simulink model "s_c107m32k_vlbi"  (R2018a)
(part 22 of 201)

      |     mask_enables{ismember(mask_names, 'sample_period')} = 'on';
      | end
      | set_param(gcb, 'MaskEnables', mask_enables);
      mask DialogControl ParameterTabVar0 Prompt: Setup
  sync_latch_hmc_wradd : Subsystem  Tag=xps:sw_reg  Commented=on  AncestorBlock=xps_library/Memory/software_register  mask(swreg){io_dir=To Processor, io_delay=0, init_val=0, sample_period=1, names=count, bitwidths=27, bin_pts=0, arith_types=0, sim_port=off, show_format=on}
      mask prompts: io_dir "I/O direction"; io_delay "I/O delay"; init_val "Initial Value"; sample_period "Sample period"; names "Bitfield names [msb...lsb]"; bitwidths "Bitfield widths"; bin_pts "Bitfield binary pts"; arith_types "Bitfield types, ufix=0, fix=1, bool=2"; sim_port "Provide sim input/output?"; show_format "Print format string?"
      mask help: A 32-bit software-accessible register. Can be divided into bitfields of varying widths and types using the fields in the block mask.
      mask init:
      | swreg_init(gcb)
      settings: AttributesFormatString=1output:uf27.0 = 27 bits
      mask TypeOptions io_dir: To Processor | From Processor
      mask Callback io_dir:
      | mask_enables = get_param(gcb, 'MaskEnables');
      | mask_names = get_param(gcb, 'MaskNames');
      | if strcmp(get_param(gcb, 'io_dir'), 'To Processor'),
      |     mask_enables{ismember(mask_names, 'sample_period')} = 'off';
      | else
      |     mask_enables{ismember(mask_names, 'sample_period')} = 'on';
      | end
      | set_param(gcb, 'MaskEnables', mask_enables);
      mask DialogControl ParameterTabVar0 Prompt: Setup
  sync_time_hmc_in_lsw : Subsystem  Tag=xps:sw_reg  Commented=on  AncestorBlock=xps_library/Memory/software_register  mask(swreg){io_dir=To Processor, io_delay=0, init_val=0, sample_period=1, names=lsw, bitwidths=32, bin_pts=0, arith_types=0, sim_port=off, show_format=on}
      mask prompts: io_dir "I/O direction"; io_delay "I/O delay"; init_val "Initial Value"; sample_period "Sample period"; names "Bitfield names [msb...lsb]"; bitwidths "Bitfield widths"; bin_pts "Bitfield binary pts"; arith_types "Bitfield types, ufix=0, fix=1, bool=2"; sim_port "Provide sim input/output?"; show_format "Print format string?"
      mask help: A 32-bit software-accessible register. Can be divided into bitfields of varying widths and types using the fields in the block mask.
      mask init:
      | swreg_init(gcb)
      settings: AttributesFormatString=1output:uf32.0 = 32 bits
      mask TypeOptions io_dir: To Processor | From Processor
      mask Callback io_dir:
      | mask_enables = get_param(gcb, 'MaskEnables');
      | mask_names = get_param(gcb, 'MaskNames');
      | if strcmp(get_param(gcb, 'io_dir'), 'To Processor'),
      |     mask_enables{ismember(mask_names, 'sample_period')} = 'off';
      | else
      |     mask_enables{ismember(mask_names, 'sample_period')} = 'on';
      | end
      | set_param(gcb, 'MaskEnables', mask_enables);
      mask DialogControl ParameterTabVar0 Prompt: Setup
  sync_time_hmc_in_msw : Subsystem  Tag=xps:sw_reg  Commented=on  AncestorBlock=xps_library/Memory/software_register  mask(swreg){io_dir=To Processor, io_delay=0, init_val=0, sample_period=1, names=msw, bitwidths=16, bin_pts=0, arith_types=0, sim_port=off, show_format=on}
      mask prompts: io_dir "I/O direction"; io_delay "I/O delay"; init_val "Initial Value"; sample_period "Sample period"; names "Bitfield names [msb...lsb]"; bitwidths "Bitfield widths"; bin_pts "Bitfield binary pts"; arith_types "Bitfield types, ufix=0, fix=1, bool=2"; sim_port "Provide sim input/output?"; show_format "Print format string?"
      mask help: A 32-bit software-accessible register. Can be divided into bitfields of varying widths and types using the fields in the block mask.
      mask init:
      | swreg_init(gcb)
      settings: AttributesFormatString=1output:uf16.0 = 16 bits
      mask TypeOptions io_dir: To Processor | From Processor
      mask Callback io_dir:
      | mask_enables = get_param(gcb, 'MaskEnables');
      | mask_names = get_param(gcb, 'MaskNames');
      | if strcmp(get_param(gcb, 'io_dir'), 'To Processor'),
      |     mask_enables{ismember(mask_names, 'sample_period')} = 'off';
      | else
      |     mask_enables{ismember(mask_names, 'sample_period')} = 'on';
      | end
      | set_param(gcb, 'MaskEnables', mask_enables);
      mask DialogControl ParameterTabVar0 Prompt: Setup
  sync_time_hmc_out_lsw : Subsystem  Tag=xps:sw_reg  Commented=on  AncestorBlock=xps_library/Memory/software_register  mask(swreg){io_dir=To Processor, io_delay=0, init_val=0, sample_period=1, names=lsw, bitwidths=32, bin_pts=0, arith_types=0, sim_port=off, show_format=on}
      mask prompts: io_dir "I/O direction"; io_delay "I/O delay"; init_val "Initial Value"; sample_period "Sample period"; names "Bitfield names [msb...lsb]"; bitwidths "Bitfield widths"; bin_pts "Bitfield binary pts"; arith_types "Bitfield types, ufix=0, fix=1, bool=2"; sim_port "Provide sim input/output?"; show_format "Print format string?"
      mask help: A 32-bit software-accessible register. Can be divided into bitfields of varying widths and types using the fields in the block mask.
      mask init:
      | swreg_init(gcb)
      settings: AttributesFormatString=1output:uf32.0 = 32 bits
      mask TypeOptions io_dir: To Processor | From Processor
      mask Callback io_dir:
      | mask_enables = get_param(gcb, 'MaskEnables');
      | mask_names = get_param(gcb, 'MaskNames');
      | if strcmp(get_param(gcb, 'io_dir'), 'To Processor'),
      |     mask_enables{ismember(mask_names, 'sample_period')} = 'off';
      | else
      |     mask_enables{ismember(mask_names, 'sample_period')} = 'on';
      | end
      | set_param(gcb, 'MaskEnables', mask_enables);
      mask DialogControl ParameterTabVar0 Prompt: Setup
  sync_time_hmc_out_msw : Subsystem  Tag=xps:sw_reg  Commented=on  AncestorBlock=xps_library/Memory/software_register  mask(swreg){io_dir=To Processor, io_delay=0, init_val=0, sample_period=1, names=msw, bitwidths=16, bin_pts=0, arith_types=0, sim_port=off, show_format=on}
      mask prompts: io_dir "I/O direction"; io_delay "I/O delay"; init_val "Initial Value"; sample_period "Sample period"; names "Bitfield names [msb...lsb]"; bitwidths "Bitfield widths"; bin_pts "Bitfield binary pts"; arith_types "Bitfield types, ufix=0, fix=1, bool=2"; sim_port "Provide sim input/output?"; show_format "Print format string?"
      mask help: A 32-bit software-accessible register. Can be divided into bitfields of varying widths and types using the fields in the block mask.
      mask init:
      | swreg_init(gcb)
      settings: AttributesFormatString=1output:uf16.0 = 16 bits
      mask TypeOptions io_dir: To Processor | From Processor
      mask Callback io_dir:
      | mask_enables = get_param(gcb, 'MaskEnables');
      | mask_names = get_param(gcb, 'MaskNames');
      | if strcmp(get_param(gcb, 'io_dir'), 'To Processor'),
      |     mask_enables{ismember(mask_names, 'sample_period')} = 'off';
      | else
      |     mask_enables{ismember(mask_names, 'sample_period')} = 'on';
      | end
      | set_param(gcb, 'MaskEnables', mask_enables);
      mask DialogControl ParameterTabVar0 Prompt: Setup
  time_gen_1 : Subsystem  Commented=on  mask{n_bits_period=0, n_bits_increment=3, n_bits_counter=48}
      mask prompts: n_bits_period "Period (2^?)"; n_bits_increment "Increment (2^?)"; n_bits_counter "Counter size (2^?)"
  time_gen_3 : Subsystem  Commented=on  mask{n_bits_period=0, n_bits_increment=3, n_bits_counter=48}
      mask prompts: n_bits_period "Period (2^?)"; n_bits_increment "Increment (2^?)"; n_bits_counter "Counter size (2^?)"
  tvg_data_gen1 : Subsystem
  tvg_data_gen_oneshot : Subsystem
      mask Display:
      | color('red');
      | disp('ONE SHOT!!');
      | % color('green');
      | % port_label('input', 1, 'dv')
      | % color('red');
      | % port_label('output', 1, 'err')
  tvg_data_tone_gen : Subsystem
  tvg_data_tone_gen1 : Subsystem
  tvg_freq_ramp_gen0 : Subsystem
  tvg_freq_ramp_gen1 : Subsystem
  tvg_time_ramp_gen0 : Subsystem
  we_delay1 : Subsystem  Tag=cmac_delinked  Commented=on  mask(pipeline){csp_latency=2}
      mask prompts: csp_latency "Latency"
      mask help:
      | An explicitly laid-out delay line to avoid mapping to SRL16s
      | for use in pipelining to help achieve timing closure.
      mask init:
      | pipeline_init(gcb,'latency',csp_latency);
      settings: AttributesFormatString=Latency = %<latency>
      mask Display:
      | port_label('input', 1, 'd');
      | port_label('output', 1, 'q');
      | disp(['Z^-', num2str(csp_latency)]);
  we_delay10 : Subsystem  Tag=cmac_delinked  Commented=on  mask(pipeline){csp_latency=2}
      mask prompts: csp_latency "Latency"
      mask help:
      | An explicitly laid-out delay line to avoid mapping to SRL16s
      | for use in pipelining to help achieve timing closure.
      mask init:
      | pipeline_init(gcb,'latency',csp_latency);
      settings: AttributesFormatString=Latency = %<latency>
      mask Display:
      | port_label('input', 1, 'd');
      | port_label('output', 1, 'q');
      | disp(['Z^-', num2str(csp_latency)]);
  we_delay11 : Subsystem  Tag=cmac_delinked  Commented=on  mask(pipeline){csp_latency=2}
      mask prompts: csp_latency "Latency"
      mask help:
      | An explicitly laid-out delay line to avoid mapping to SRL16s
      | for use in pipelining to help achieve timing closure.
      mask init:
      | pipeline_init(gcb,'latency',csp_latency);
      settings: AttributesFormatString=Latency = %<latency>
      mask Display:
      | port_label('input', 1, 'd');
      | port_label('output', 1, 'q');
      | disp(['Z^-', num2str(csp_latency)]);
  we_delay12 : Subsystem  Tag=cmac_delinked  Commented=on  mask(pipeline){csp_latency=2}
      mask prompts: csp_latency "Latency"
      mask help:
      | An explicitly laid-out delay line to avoid mapping to SRL16s
      | for use in pipelining to help achieve timing closure.
      mask init:
      | pipeline_init(gcb,'latency',csp_latency);
      settings: AttributesFormatString=Latency = %<latency>
      mask Display:
      | port_label('input', 1, 'd');
      | port_label('output', 1, 'q');
      | disp(['Z^-', num2str(csp_latency)]);
  we_delay13 : Subsystem  Tag=cmac_delinked  Commented=on  mask(pipeline){csp_latency=2}
      mask prompts: csp_latency "Latency"
      mask help:
      | An explicitly laid-out delay line to avoid mapping to SRL16s
      | for use in pipelining to help achieve timing closure.
      mask init:
      | pipeline_init(gcb,'latency',csp_latency);
      settings: AttributesFormatString=Latency = %<latency>
      mask Display:
      | port_label('input', 1, 'd');
      | port_label('output', 1, 'q');
      | disp(['Z^-', num2str(csp_latency)]);
  we_delay14 : Subsystem  Tag=cmac_delinked  Commented=on  mask(pipeline){csp_latency=2}
      mask prompts: csp_latency "Latency"
      mask help:
      | An explicitly laid-out delay line to avoid mapping to SRL16s
      | for use in pipelining to help achieve timing closure.
      mask init:
      | pipeline_init(gcb,'latency',csp_latency);
      settings: AttributesFormatString=Latency = %<latency>
      mask Display:
      | port_label('input', 1, 'd');
      | port_label('output', 1, 'q');
      | disp(['Z^-', num2str(csp_latency)]);
  we_delay15 : Subsystem  Tag=cmac_delinked  Commented=on  mask(pipeline){csp_latency=2}
      mask prompts: csp_latency "Latency"
      mask help:
      | An explicitly laid-out delay line to avoid mapping to SRL16s
      | for use in pipelining to help achieve timing closure.
      mask init:
      | pipeline_init(gcb,'latency',csp_latency);
      settings: AttributesFormatString=Latency = %<latency>
      mask Display:
      | port_label('input', 1, 'd');
      | port_label('output', 1, 'q');
      | disp(['Z^-', num2str(csp_latency)]);
  we_delay16 : Subsystem  Tag=cmac_delinked  Commented=on  mask(pipeline){csp_latency=2}
      mask prompts: csp_latency "Latency"
      mask help:
      | An explicitly laid-out delay line to avoid mapping to SRL16s
      | for use in pipelining to help achieve timing closure.
      mask init:
      | pipeline_init(gcb,'latency',csp_latency);
      settings: AttributesFormatString=Latency = %<latency>
      mask Display:
      | port_label('input', 1, 'd');
      | port_label('output', 1, 'q');
      | disp(['Z^-', num2str(csp_latency)]);
  we_delay17 : Subsystem  Tag=cmac_delinked  Commented=on  mask(pipeline){csp_latency=2}
      mask prompts: csp_latency "Latency"
      mask help:
      | An explicitly laid-out delay line to avoid mapping to SRL16s
      | for use in pipelining to help achieve timing closure.
      mask init:
      | pipeline_init(gcb,'latency',csp_latency);
      settings: AttributesFormatString=Latency = %<latency>
      mask Display:
      | port_label('input', 1, 'd');
      | port_label('output', 1, 'q');
      | disp(['Z^-', num2str(csp_latency)]);
  we_delay18 : Subsystem  Tag=cmac_delinked  Commented=on  mask(pipeline){csp_latency=2}
      mask prompts: csp_latency "Latency"
      mask help:
      | An explicitly laid-out delay line to avoid mapping to SRL16s
      | for use in pipelining to help achieve timing closure.
      mask init:
      | pipeline_init(gcb,'latency',csp_latency);
      settings: AttributesFormatString=Latency = %<latency>
      mask Display:
      | port_label('input', 1, 'd');
      | port_label('output', 1, 'q');
      | disp(['Z^-', num2str(csp_latency)]);
  we_delay19 : Subsystem  Tag=cmac_delinked  Commented=on  mask(pipeline){csp_latency=2}
      mask prompts: csp_latency "Latency"
      mask help:
      | An explicitly laid-out delay line to avoid mapping to SRL16s
      | for use in pipelining to help achieve timing closure.
      mask init:
      | pipeline_init(gcb,'latency',csp_latency);
      settings: AttributesFormatString=Latency = %<latency>
      mask Display:
      | port_label('input', 1, 'd');
      | port_label('output', 1, 'q');
      | disp(['Z^-', num2str(csp_latency)]);
  we_delay2 : Subsystem  Tag=cmac_delinked  Commented=on  mask(pipeline){csp_latency=2}
      mask prompts: csp_latency "Latency"
      mask help:
      | An explicitly laid-out delay line to avoid mapping to SRL16s
      | for use in pipelining to help achieve timing closure.
      mask init:
      | pipeline_init(gcb,'latency',csp_latency);
      settings: AttributesFormatString=Latency = %<latency>
      mask Display:
      | port_label('input', 1, 'd');
      | port_label('output', 1, 'q');
      | disp(['Z^-', num2str(csp_latency)]);
  we_delay20 : Subsystem  Tag=cmac_delinked  Commented=on  mask(pipeline){csp_latency=2}
      mask prompts: csp_latency "Latency"
      mask help:
      | An explicitly laid-out delay line to avoid mapping to SRL16s
      | for use in pipelining to help achieve timing closure.
      mask init:
      | pipeline_init(gcb,'latency',csp_latency);
      settings: AttributesFormatString=Latency = %<latency>
      mask Display:
      | port_label('input', 1, 'd');
      | port_label('output', 1, 'q');
      | disp(['Z^-', num2str(csp_latency)]);
  we_delay21 : Subsystem  Tag=cmac_delinked  Commented=on  mask(pipeline){csp_latency=2}
      mask prompts: csp_latency "Latency"
      mask help:
      | An explicitly laid-out delay line to avoid mapping to SRL16s
      | for use in pipelining to help achieve timing closure.
      mask init:
      | pipeline_init(gcb,'latency',csp_latency);
      settings: AttributesFormatString=Latency = %<latency>
      mask Display:
      | port_label('input', 1, 'd');
      | port_label('output', 1, 'q');
      | disp(['Z^-', num2str(csp_latency)]);
  we_delay22 : Subsystem  Tag=cmac_delinked  Commented=on  mask(pipeline){csp_latency=2}
      mask prompts: csp_latency "Latency"
      mask help:
      | An explicitly laid-out delay line to avoid mapping to SRL16s
      | for use in pipelining to help achieve timing closure.
      mask init:
      | pipeline_init(gcb,'latency',csp_latency);
      settings: AttributesFormatString=Latency = %<latency>
      mask Display:
      | port_label('input', 1, 'd');
      | port_label('output', 1, 'q');
      | disp(['Z^-', num2str(csp_latency)]);
  we_delay23 : Subsystem  Tag=cmac_delinked  Commented=on  mask(pipeline){csp_latency=2}
      mask prompts: csp_latency "Latency"
      mask help:
      | An explicitly laid-out delay line to avoid mapping to SRL16s
      | for use in pipelining to help achieve timing closure.
      mask init:
      | pipeline_init(gcb,'latency',csp_latency);
      settings: AttributesFormatString=Latency = %<latency>
      mask Display:
      | port_label('input', 1, 'd');
      | port_label('output', 1, 'q');
      | disp(['Z^-', num2str(csp_latency)]);
  we_delay24 : Subsystem  Tag=cmac_delinked  Commented=on  mask(pipeline){csp_latency=2}
      mask prompts: csp_latency "Latency"
      mask help:
      | An explicitly laid-out delay line to avoid mapping to SRL16s
      | for use in pipelining to help achieve timing closure.
      mask init:
      | pipeline_init(gcb,'latency',csp_latency);
      settings: AttributesFormatString=Latency = %<latency>
      mask Display:
      | port_label('input', 1, 'd');
      | port_label('output', 1, 'q');
      | disp(['Z^-', num2str(csp_latency)]);
  we_delay25 : Subsystem  Tag=cmac_delinked  Commented=on  mask(pipeline){csp_latency=2}
      mask prompts: csp_latency "Latency"
      mask help:
      | An explicitly laid-out delay line to avoid mapping to SRL16s
      | for use in pipelining to help achieve timing closure.
      mask init:
      | pipeline_init(gcb,'latency',csp_latency);
      settings: AttributesFormatString=Latency = %<latency>
      mask Display:
      | port_label('input', 1, 'd');
      | port_label('output', 1, 'q');
      | disp(['Z^-', num2str(csp_latency)]);
  we_delay26 : Subsystem  Tag=cmac_delinked  Commented=on  mask(pipeline){csp_latency=2}
      mask prompts: csp_latency "Latency"
      mask help:
      | An explicitly laid-out delay line to avoid mapping to SRL16s
      | for use in pipelining to help achieve timing closure.
      mask init:
      | pipeline_init(gcb,'latency',csp_latency);
      settings: AttributesFormatString=Latency = %<latency>
      mask Display:
      | port_label('input', 1, 'd');
      | port_label('output', 1, 'q');
      | disp(['Z^-', num2str(csp_latency)]);
  we_delay27 : Subsystem  Tag=cmac_delinked  Commented=on  mask(pipeline){csp_latency=2}
      mask prompts: csp_latency "Latency"
      mask help:
      | An explicitly laid-out delay line to avoid mapping to SRL16s
      | for use in pipelining to help achieve timing closure.
      mask init:
      | pipeline_init(gcb,'latency',csp_latency);
      settings: AttributesFormatString=Latency = %<latency>
      mask Display:
      | port_label('input', 1, 'd');
      | port_label('output', 1, 'q');
      | disp(['Z^-', num2str(csp_latency)]);
  we_delay28 : Subsystem  Tag=cmac_delinked  Commented=on  mask(pipeline){csp_latency=2}
      mask prompts: csp_latency "Latency"
      mask help:
      | An explicitly laid-out delay line to avoid mapping to SRL16s
      | for use in pipelining to help achieve timing closure.
      mask init:
      | pipeline_init(gcb,'latency',csp_latency);
      settings: AttributesFormatString=Latency = %<latency>
      mask Display:
      | port_label('input', 1, 'd');
      | port_label('output', 1, 'q');
      | disp(['Z^-', num2str(csp_latency)]);
  we_delay29 : Subsystem  Tag=cmac_delinked  Commented=on  mask(pipeline){csp_latency=2}
      mask prompts: csp_latency "Latency"
      mask help:
      | An explicitly laid-out delay line to avoid mapping to SRL16s
      | for use in pipelining to help achieve timing closure.
      mask init:
      | pipeline_init(gcb,'latency',csp_latency);
      settings: AttributesFormatString=Latency = %<latency>
      mask Display:
      | port_label('input', 1, 'd');
      | port_label('output', 1, 'q');
      | disp(['Z^-', num2str(csp_latency)]);
  we_delay3 : Subsystem  Tag=cmac_delinked  Commented=on  mask(pipeline){csp_latency=2}
      mask prompts: csp_latency "Latency"
      mask help:
      | An explicitly laid-out delay line to avoid mapping to SRL16s
      | for use in pipelining to help achieve timing closure.
      mask init:
      | pipeline_init(gcb,'latency',csp_latency);
      settings: AttributesFormatString=Latency = %<latency>
      mask Display:
      | port_label('input', 1, 'd');
      | port_label('output', 1, 'q');
      | disp(['Z^-', num2str(csp_latency)]);
  we_delay30 : Subsystem  Tag=cmac_delinked  Commented=on  mask(pipeline){csp_latency=2}
      mask prompts: csp_latency "Latency"
      mask help:
      | An explicitly laid-out delay line to avoid mapping to SRL16s
      | for use in pipelining to help achieve timing closure.
      mask init:
      | pipeline_init(gcb,'latency',csp_latency);
      settings: AttributesFormatString=Latency = %<latency>
      mask Display:
      | port_label('input', 1, 'd');
      | port_label('output', 1, 'q');
      | disp(['Z^-', num2str(csp_latency)]);
  we_delay31 : Subsystem  Tag=cmac_delinked  Commented=on  mask(pipeline){csp_latency=2}
      mask prompts: csp_latency "Latency"
      mask help:
      | An explicitly laid-out delay line to avoid mapping to SRL16s
      | for use in pipelining to help achieve timing closure.
      mask init:
      | pipeline_init(gcb,'latency',csp_latency);
      settings: AttributesFormatString=Latency = %<latency>
      mask Display:
      | port_label('input', 1, 'd');
      | port_label('output', 1, 'q');
      | disp(['Z^-', num2str(csp_latency)]);
  we_delay32 : Subsystem  Tag=cmac_delinked  Commented=on  mask(pipeline){csp_latency=2}
      mask prompts: csp_latency "Latency"
      mask help:
      | An explicitly laid-out delay line to avoid mapping to SRL16s
      | for use in pipelining to help achieve timing closure.
      mask init:
      | pipeline_init(gcb,'latency',csp_latency);
      settings: AttributesFormatString=Latency = %<latency>
      mask Display:
      | port_label('input', 1, 'd');
      | port_label('output', 1, 'q');
      | disp(['Z^-', num2str(csp_latency)]);
  we_delay33 : Subsystem  Tag=cmac_delinked  Commented=on  mask(pipeline){csp_latency=2}
      mask prompts: csp_latency "Latency"
      mask help:
      | An explicitly laid-out delay line to avoid mapping to SRL16s
      | for use in pipelining to help achieve timing closure.
      mask init:
      | pipeline_init(gcb,'latency',csp_latency);
      settings: AttributesFormatString=Latency = %<latency>
      mask Display:
      | port_label('input', 1, 'd');
      | port_label('output', 1, 'q');
      | disp(['Z^-', num2str(csp_latency)]);
  we_delay34 : Subsystem  Tag=cmac_delinked  Commented=on  mask(pipeline){csp_latency=2}
      mask prompts: csp_latency "Latency"
      mask help:
      | An explicitly laid-out delay line to avoid mapping to SRL16s
      | for use in pipelining to help achieve timing closure.
      mask init:
      | pipeline_init(gcb,'latency',csp_latency);
      settings: AttributesFormatString=Latency = %<latency>
      mask Display:
      | port_label('input', 1, 'd');
      | port_label('output', 1, 'q');
      | disp(['Z^-', num2str(csp_latency)]);
  we_delay35 : Subsystem  Tag=cmac_delinked  Commented=on  mask(pipeline){csp_latency=2}
      mask prompts: csp_latency "Latency"
      mask help:
      | An explicitly laid-out delay line to avoid mapping to SRL16s
      | for use in pipelining to help achieve timing closure.
      mask init:
      | pipeline_init(gcb,'latency',csp_latency);
      settings: AttributesFormatString=Latency = %<latency>
      mask Display:
      | port_label('input', 1, 'd');
      | port_label('output', 1, 'q');
      | disp(['Z^-', num2str(csp_latency)]);
  we_delay36 : Subsystem  Tag=cmac_delinked  Commented=on  mask(pipeline){csp_latency=2}
      mask prompts: csp_latency "Latency"
      mask help:
      | An explicitly laid-out delay line to avoid mapping to SRL16s
      | for use in pipelining to help achieve timing closure.
      mask init:
      | pipeline_init(gcb,'latency',csp_latency);
      settings: AttributesFormatString=Latency = %<latency>
      mask Display:
      | port_label('input', 1, 'd');
      | port_label('output', 1, 'q');
      | disp(['Z^-', num2str(csp_latency)]);
  we_delay37 : Subsystem  Tag=cmac_delinked  Commented=on  mask(pipeline){csp_latency=2}
      mask prompts: csp_latency "Latency"
      mask help:
      | An explicitly laid-out delay line to avoid mapping to SRL16s
      | for use in pipelining to help achieve timing closure.
      mask init:
      | pipeline_init(gcb,'latency',csp_latency);
      settings: AttributesFormatString=Latency = %<latency>
      mask Display:
      | port_label('input', 1, 'd');
      | port_label('output', 1, 'q');
      | disp(['Z^-', num2str(csp_latency)]);
  we_delay38 : Subsystem  Tag=cmac_delinked  Commented=on  mask(pipeline){csp_latency=2}
      mask prompts: csp_latency "Latency"
      mask help:
      | An explicitly laid-out delay line to avoid mapping to SRL16s
      | for use in pipelining to help achieve timing closure.
      mask init:
      | pipeline_init(gcb,'latency',csp_latency);
      settings: AttributesFormatString=Latency = %<latency>
      mask Display:
      | port_label('input', 1, 'd');
      | port_label('output', 1, 'q');
      | disp(['Z^-', num2str(csp_latency)]);
  we_delay39 : Subsystem  Tag=cmac_delinked  Commented=on  mask(pipeline){csp_latency=2}
      mask prompts: csp_latency "Latency"
      mask help:
      | An explicitly laid-out delay line to avoid mapping to SRL16s
      | for use in pipelining to help achieve timing closure.
      mask init:
      | pipeline_init(gcb,'latency',csp_latency);
      settings: AttributesFormatString=Latency = %<latency>
      mask Display:
      | port_label('input', 1, 'd');
      | port_label('output', 1, 'q');
      | disp(['Z^-', num2str(csp_latency)]);
  we_delay4 : Subsystem  Tag=cmac_delinked  Commented=on  mask(pipeline){csp_latency=2}
      mask prompts: csp_latency "Latency"
      mask help:
      | An explicitly laid-out delay line to avoid mapping to SRL16s
      | for use in pipelining to help achieve timing closure.
      mask init:
      | pipeline_init(gcb,'latency',csp_latency);
      settings: AttributesFormatString=Latency = %<latency>
      mask Display:
      | port_label('input', 1, 'd');
      | port_label('output', 1, 'q');
      | disp(['Z^-', num2str(csp_latency)]);
  we_delay5 : Subsystem  Tag=cmac_delinked  Commented=on  mask(pipeline){csp_latency=2}
      mask prompts: csp_latency "Latency"
      mask help:
      | An explicitly laid-out delay line to avoid mapping to SRL16s
      | for use in pipelining to help achieve timing closure.
      mask init:
      | pipeline_init(gcb,'latency',csp_latency);
      settings: AttributesFormatString=Latency = %<latency>
      mask Display:
      | port_label('input', 1, 'd');
      | port_label('output', 1, 'q');
      | disp(['Z^-', num2str(csp_latency)]);
  we_delay53 : Subsystem  Tag=cmac_delinked  Commented=on  mask(pipeline){csp_latency=2}
      mask prompts: csp_latency "Latency"
      mask help:
      | An explicitly laid-out delay line to avoid mapping to SRL16s
      | for use in pipelining to help achieve timing closure.
      mask init:
      | pipeline_init(gcb,'latency',csp_latency);
      settings: AttributesFormatString=Latency = %<latency>
      mask Display:
      | port_label('input', 1, 'd');
      | port_label('output', 1, 'q');
      | disp(['Z^-', num2str(csp_latency)]);
  we_delay6 : Subsystem  Tag=cmac_delinked  Commented=on  mask(pipeline){csp_latency=2}
      mask prompts: csp_latency "Latency"
      mask help:
      | An explicitly laid-out delay line to avoid mapping to SRL16s
      | for use in pipelining to help achieve timing closure.
      mask init:
      | pipeline_init(gcb,'latency',csp_latency);
      settings: AttributesFormatString=Latency = %<latency>
      mask Display:
      | port_label('input', 1, 'd');
      | port_label('output', 1, 'q');
      | disp(['Z^-', num2str(csp_latency)]);
  we_delay66 : Subsystem  Tag=cmac_delinked  Commented=on  mask(pipeline){csp_latency=2}
      mask prompts: csp_latency "Latency"
      mask help:
      | An explicitly laid-out delay line to avoid mapping to SRL16s
      | for use in pipelining to help achieve timing closure.
      mask init:
      | pipeline_init(gcb,'latency',csp_latency);
      settings: AttributesFormatString=Latency = %<latency>
      mask Display:
      | port_label('input', 1, 'd');
      | port_label('output', 1, 'q');
      | disp(['Z^-', num2str(csp_latency)]);
  we_delay7 : Subsystem  Tag=cmac_delinked  Commented=on  mask(pipeline){csp_latency=2}
      mask prompts: csp_latency "Latency"
      mask help:
      | An explicitly laid-out delay line to avoid mapping to SRL16s
      | for use in pipelining to help achieve timing closure.
      mask init:
      | pipeline_init(gcb,'latency',csp_latency);
      settings: AttributesFormatString=Latency = %<latency>
      mask Display:
      | port_label('input', 1, 'd');
      | port_label('output', 1, 'q');
      | disp(['Z^-', num2str(csp_latency)]);
  we_delay8 : Subsystem  Tag=cmac_delinked  Commented=on  mask(pipeline){csp_latency=2}
      mask prompts: csp_latency "Latency"
      mask help:
      | An explicitly laid-out delay line to avoid mapping to SRL16s
      | for use in pipelining to help achieve timing closure.
      mask init:
      | pipeline_init(gcb,'latency',csp_latency);
      settings: AttributesFormatString=Latency = %<latency>
      mask Display:
      | port_label('input', 1, 'd');
      | port_label('output', 1, 'q');
      | disp(['Z^-', num2str(csp_latency)]);
  we_delay9 : Subsystem  Tag=cmac_delinked  Commented=on  mask(pipeline){csp_latency=2}
      mask prompts: csp_latency "Latency"
      mask help:
      | An explicitly laid-out delay line to avoid mapping to SRL16s
      | for use in pipelining to help achieve timing closure.
      mask init:
      | pipeline_init(gcb,'latency',csp_latency);
      settings: AttributesFormatString=Latency = %<latency>
      mask Display:
      | port_label('input', 1, 'd');
      | port_label('output', 1, 'q');
      | disp(['Z^-', num2str(csp_latency)]);
  xeng_match : Subsystem  Tag=xps:sw_reg  AncestorBlock=xps_library/Memory/software_register  mask(swreg){io_dir=From Processor, io_delay=0, init_val=0, sample_period=1, names=[val], bitwidths=[3], bin_pts=0, arith_types=0, sim_port=on, show_format=on}
      mask prompts: io_dir "I/O direction"; io_delay "I/O delay"; init_val "Initial Value"; sample_period "Sample period"; names "Bitfield names [msb...lsb]"; bitwidths "Bitfield widths"; bin_pts "Bitfield binary pts"; arith_types "Bitfield types, ufix=0, fix=1, bool=2"; sim_port "Provide sim input/output?"; show_format "Print format string?"
      mask help: A 32-bit software-accessible register. Can be divided into bitfields of varying widths and types using the fields in the block mask.
      mask init:
      | swreg_init(gcb)
      settings: AttributesFormatString=1input:uf3.0 = 3 bits
      mask TypeOptions io_dir: To Processor | From Processor
      mask Callback io_dir:
      | mask_enables = get_param(gcb, 'MaskEnables');
      | mask_names = get_param(gcb, 'MaskNames');
      | if strcmp(get_param(gcb, 'io_dir'), 'To Processor'),
      |     mask_enables{ismember(mask_names, 'sample_period')} = 'off';
      | else
      |     mask_enables{ismember(mask_names, 'sample_period')} = 'on';
      | end
      | set_param(gcb, 'MaskEnables', mask_enables);
      mask DialogControl ParameterTabVar0 Prompt: Setup
  xidx_trig_thresh : Subsystem  Tag=xps:sw_reg  AncestorBlock=xps_library/Memory/software_register  mask(swreg){io_dir=From Processor, io_delay=0, init_val=0, sample_period=1, names=[threshold], bitwidths=[15], bin_pts=0, arith_types=0, sim_port=on, show_format=on}
      mask prompts: io_dir "I/O direction"; io_delay "I/O delay"; init_val "Initial Value"; sample_period "Sample period"; names "Bitfield names [msb...lsb]"; bitwidths "Bitfield widths"; bin_pts "Bitfield binary pts"; arith_types "Bitfield types, ufix=0, fix=1, bool=2"; sim_port "Provide sim input/output?"; show_format "Print format string?"
      mask help: A 32-bit software-accessible register. Can be divided into bitfields of varying widths and types using the fields in the block mask.
      mask init:
      | swreg_init(gcb)
      settings: AttributesFormatString=1input:uf15.0 = 15 bits
      mask TypeOptions io_dir: To Processor | From Processor
      mask Callback io_dir:
      | mask_enables = get_param(gcb, 'MaskEnables');
      | mask_names = get_param(gcb, 'MaskNames');
      | if strcmp(get_param(gcb, 'io_dir'), 'To Processor'),
      |     mask_enables{ismember(mask_names, 'sample_period')} = 'off';
      | else
      |     mask_enables{ismember(mask_names, 'sample_period')} = 'on';
      | end
      | set_param(gcb, 'MaskEnables', mask_enables);
      mask DialogControl ParameterTabVar0 Prompt: Setup
  out_sync : Outport
  out_dv : Outport  Port=2
  out_d256 : Outport  Port=3
  pkt_start : Outport  Port=4
  freq_id : Outport  Port=5
  x_index : Outport  Port=6
  x_pkt_index : Outport  Port=7
  error0 : Outport  Port=8
  tvg_error : Outport  Port=9
  tag scope: cthmc_sync_err_g0=global, hmc_sync_g=global, raw_freq_ctr_g=global, rd_addr_final_g0=global, rd_addr_final_g1=global, rd_en_final_g0=global, rd_en_final_g1=global, rd_tag_final_g0=global, wr_addr_final_g0=global, wr_addr_final_g1=global, wr_data_final_g0=global, wr_data_final_g1=global, wr_en_final_g0=global, wr_en_final_g1=global
  wires:
  Delay6/1 -> Subsystem1/2(en), Delay26/1
  Delay10/1 -> Delay27/1
  Delay16/1 -> Delay28/1
  Delay9/1 -> spectrum_ctr2/1, spectrum_ctr3/1
  [hmc_sync] -> Delay5/1
  [hmc_dv_0] -> Delay7/1
  [hmc_tag_0] -> Delay8/1
  [ct_tag_insert_sel] -> Mux/1
  [hmc_d256_0] -> spectrum_ctr4/1
  spectrum_ctr4/1 -> Mux/2
  [hmc_tag_0] -> Mux/3
  Concat13/1 -> obuf/4(din0)
  spectrum_ctr3/1 -> Concat13/3
  Mux/1 -> Concat13/2
  spectrum_ctr2/1 -> Concat13/1
  Delay8/1 -> obuf/3(tag0)
  Delay7/1 -> obuf/2(dv0)
  Delay5/1 -> obuf/1(sync)
  obuf/4(pkt_start) -> Delay16/1
  obuf/2(out_dv) -> Delay6/1, gen_freq_calc/2(dv)
  in_d0/1 -> Delay34/1
  [ct_tvg_en] -> Mux3/1
  Delay35/1 -> Delay15/1, Gateway Out/1, Counter/1
  Concat3/1 -> Delay42/1
  Mux3/1 -> Concat3/4, Delay46/1  "data128"
  in_dv/1 -> Logical7/2, Delay33/1, tvg_data_gen_oneshot/2(dv), tvg_data_tone_gen1/2(dv), tvg_freq_ramp_gen1/2(dv), tvg_data_tone_gen/2(dv), tvg_data_gen1/2(dv), tvg_freq_ramp_gen0/2(dv), tvg_time_ramp_gen0/2(dv)  "dv128"
  in_sync/1 -> Counter45/1, Register36/2, Register17/2, Counter2/1, Register3/1, Register3/3, Register9/2, tvg_data_gen_oneshot/1(sync), tvg_data_tone_gen1/1(sync), tvg_freq_ramp_gen1/1(sync), tvg_data_tone_gen/1(sync), tvg_data_gen1/1(sync), tvg_freq_ramp_gen0/1(sync), tvg_time_ramp_gen0/1(sync), Delay36/1  "sync128"
  Delay33/1 -> Delay39/1
  Delay36/1 -> Delay35/1
  [rd_addr_arm_raw] -> Inverter6/1
  [sync256] -> Logical15/1
  Inverter6/1 -> Logical15/2
  Logical15/1 -> [cthmc_sync_err_g0]
  [tvgtone_p1] -> tvg_data_tone_gen/3(target)
  [tvgtone_level1] -> tvg_data_tone_gen/4(level)
  Delay15/1 -> Delay44/1, Delay84/1, Delay80/1  "sync256"
  Delay42/1 -> Delay43/1, Delay14/1  "d256"
  Delay1/1 -> Delay45/1, Delay77/1, Delay81/2, Delay82/1, Delay14/2  "dv_256"
  Delay45/1 -> [dv256], Terminator/1  "ORIG"
  Delay43/1 -> [d256_0]
  Delay44/1 -> [sync256]
  Delay34/1 -> Mux3/2
  [wr_addr] -> [wr_addr_0]
  [rd_addr] -> [rd_addr_1]
  [rd_tag] -> [rd_tag_0]
  Logical5/1 -> hmc/1, [wr_en_final_g0]
  [wr_en_0] -> Logical5/2  "WR_en"
  Logical11/1 -> hmc/4, [rd_en_final_g0]
  [rd_en_0] -> Logical11/2  "RD_en"
  pipeline1/1(q) -> hmc/3, [wr_data_final_g0]
  pipeline2/1(q) -> hmc/5, [rd_addr_final_g0]
  pipeline3/1(q) -> hmc/6, [rd_tag_final_g0]
  [wr_addr_final_g0] -> Slice12/1
  [rd_addr_final_g0] -> Slice13/1
  Slice13/1 -> Logical/2  "final_rd_bank"
  Slice12/1 -> Logical/1  "final_wr_bank"
  Logical/1 -> Logical8/1
  Logical10/1 -> Logical8/2
  [wr_en_final_g0] -> Logical10/1
  [rd_en_final_g0] -> Logical10/2
  Logical8/1 -> [ct_bank_error_g0]  "same_bank"
  hmc/5 -> pipeline6/1(d)
  hmc/4 -> [hmc_rd_rdy_0]
  hmc/3 -> [hmc_wr_rdy_0]
  convert_rd_en4/1 -> pipeline5/1(d)  "hmcout_dv"
  pipeline6/1(q) -> [hmc_tag_0_tmp]  "hmc_tag"
  pipeline5/1(q) -> [hmc_dv_0_tmp]  "hmc_dv"
  pipeline4/1(q) -> [hmc_d256_0_tmp]
  hmc/1 -> pipeline4/1(d)  "hmc_d256"
  hmc/2 -> convert_rd_en4/1
  [rd_addr_arm] -> edge_detect1/1(in)
  edge_detect1/1(out) -> [hmc_sync_tmp]
  [hmc_ok0] -> Logical11/1, Logical5/1
  pipeline/1(q) -> [wr_addr_final_g0], hmc/2
  [wr_addr_final_g1] -> Slice8/1
  [rd_addr_final_g1] -> Slice9/1
  Slice9/1 -> Logical19/2  "final_rd_bank"
  Slice8/1 -> Logical19/1  "final_wr_bank"
  Logical19/1 -> Logical21/1
  Logical20/1 -> Logical21/2
  [wr_en_final_g1] -> Logical20/1
  [rd_en_final_g1] -> Logical20/2
  Logical21/1 -> [ct_bank_error_g1]  "same_bank"
  Constant/1 -> hmc/7
  Constant1/1 -> hmc/8
  Constant2/1 -> hmc/9
  Constant3/1 -> hmc/10
  Constant4/1 -> hmc/11
  Constant5/1 -> hmc/12
  hmc/7 -> Terminator2/1
  hmc/6 -> Terminator1/1
  hmc/8 -> Terminator3/1
  hmc/9 -> Terminator4/1
  hmc/10 -> Terminator5/1
  [rd_tag_1] -> pipeline13/1(d)  "RD_tag"
  [wr_addr_1] -> pipeline10/1(d)  "WR_addr"
  [wr_d256_1] -> pipeline11/1(d)
  [rd_addr_1] -> pipeline12/1(d)  "RD_rdaddr"
  Logical18/1 -> [wr_en_final_g1], hmc1/1
  [wr_en_1] -> Logical18/2  "WR_en"
  Logical2/1 -> [rd_en_final_g1], hmc1/4
  [rd_en_1] -> Logical2/2  "RD_en"
  pipeline11/1(q) -> [wr_data_final_g1], hmc1/3
  pipeline12/1(q) -> [rd_addr_final_g1], hmc1/5
  pipeline13/1(q) -> hmc1/6
  hmc1/5 -> pipeline9/1(d)
  hmc1/4 -> [hmc_rd_rdy_1]
  hmc1/3 -> [hmc_wr_rdy_1]
  convert_rd_en1/1 -> pipeline8/1(d)  "hmcout_dv"
  pipeline8/1(q) -> [hmc_dv_1_tmp]  "hmc_dv"
  pipeline7/1(q) -> [hmc_d256_1_tmp]
  hmc1/1 -> pipeline7/1(d)  "hmc_d256"
  hmc1/2 -> convert_rd_en1/1
  [hmc_ok1] -> Logical2/1, Logical18/1
  pipeline10/1(q) -> hmc1/2, [wr_addr_final_g1]
  Constant6/1 -> hmc1/7
  Constant7/1 -> hmc1/8
  Constant8/1 -> hmc1/9
  Constant9/1 -> hmc1/10
  Constant10/1 -> hmc1/11
  Constant11/1 -> hmc1/12
  hmc1/7 -> Terminator11/1
  hmc1/6 -> Terminator10/1
  hmc1/8 -> Terminator12/1
  hmc1/9 -> Terminator13/1
  hmc1/10 -> Terminator14/1
  [sync256] -> hmc_addr_gen/1(sync)
  [d256_0] -> hmc_addr_gen/3(d256_0)
  hmc_addr_gen/1(wr_sync) -> [wr_sync]
  hmc_addr_gen/10(rd_arm_raw) -> [rd_addr_arm_raw]
  [hmc_sync_tmp] -> Delay89/1
  Delay89/1 -> Delay93/1, [hmc_sync_g]
  [hmc_d256_0_tmp] -> Delay90/1
  Delay90/1 -> [hmc_d256_0]
  [hmc_dv_0_tmp] -> Delay2/1
  Delay2/1 -> [hmc_dv_0]
  [hmc_tag_0_tmp] -> Delay3/1
  Delay3/1 -> [hmc_tag_0]
  Delay93/1 -> [hmc_sync]
  gen_freq_calc/1(raw_ctr64) -> Delay29/1
  gen_freq_calc/2(freq) -> Subsystem1/4(frequency), Delay40/1
  gen_freq_calc/3(x_index) -> Delay61/1
  gen_freq_calc/4(x_pkt_index) -> Delay62/1
  [ct_freq_gen_offset] -> gen_freq_calc/3(freq_offset)
  pipeline9/1(q) -> [hmc_tag_1_tmp]  "hmc_tag"
  [hmc_wr_rdy_0] -> Inverter1/1
  [hmc_rd_rdy_0] -> Inverter2/1
  [hmc_wr_rdy_1] -> Inverter22/1
  [hmc_rd_rdy_1] -> Inverter23/1
  Logical4/1 -> error0/1
  [ct_tvg_en] -> Mux4/1
  tvg_data_tone_gen/1(d) -> Mux4/4
  Delay41/1 -> Mux4/2
  in_d1/1 -> Delay41/1
  Delay46/1 -> Concat3/3, Delay47/1
  Delay47/1 -> Concat3/2, Delay51/1
  Delay51/1 -> Concat3/1
  Constant12/1 -> Relational/2
  Counter/1 -> Gateway Out2/1, Relational/1
  Relational/1 -> Logical1/1
  Gateway Out/1 -> Scope/1
  Gateway Out1/1 -> Scope/2
  Gateway Out2/1 -> Scope/3
  Gateway Out3/1 -> Scope/4
  Concat2/1 -> Delay78/1
  Mux4/1 -> Concat2/4, Delay60/1  "data128"
  Delay60/1 -> Delay64/1, Concat2/3
  Delay64/1 -> Delay65/1, Concat2/2
  Delay65/1 -> Concat2/1
  Delay75/1 -> [d256_1]
  Delay78/1 -> Delay75/1, Delay81/1
  [dv256] -> hmc_addr_gen/2(dv)
  [d256_1] -> hmc_addr_gen/4(d256_1)
  hmc_addr_gen/2(wr_en) -> [wr_en]
  hmc_addr_gen/3(wr_addr) -> [wr_addr]
  hmc_addr_gen/4(wr_d256_0) -> [wr_d256_0]
  hmc_addr_gen/5(wr_d256_1) -> [wr_d256_1]
  hmc_addr_gen/6(rd_en) -> [rd_en]
  hmc_addr_gen/8(rd_tag) -> [rd_tag]
  hmc_addr_gen/7(rd_addr) -> [rd_addr]
  hmc_addr_gen/9(rd_addr_arm) -> [rd_addr_arm]
  [rd_en] -> [rd_en_0]
  tvg_data_gen1/1(d) -> Mux4/3
  tvg_time_ramp_gen0/1(d) -> Mux3/3
  tvg_freq_ramp_gen0/1(d) -> Mux3/5
  tvg_freq_ramp_gen1/1(d) -> Mux4/5
  Gateway Out8/1 -> Scope2/1
  Gateway Out9/1 -> Scope2/2
  Gateway Out10/1 -> Scope2/3
  Gateway Out11/1 -> Scope2/4
  Delay39/1 -> Gateway Out1/1, Counter/2, Delay54/1, Delay60/2, Delay64/2, Delay65/2, Delay46/2, Delay47/2, Delay51/2, Logical1/2
  Delay54/1 -> Delay83/1, Delay79/1
  Slice/1 -> Gateway Out11/1
  [tvgtone_p0] -> tvg_data_tone_gen1/3(target)
  [tvgtone_level0] -> tvg_data_tone_gen1/4(level)
  tvg_data_tone_gen1/1(d) -> Mux3/4
  Logical1/1 -> Delay1/1, Gateway Out3/1
  Delay14/1 -> Slice/1
  Delay77/1 -> Gateway Out10/1
  Delay79/1 -> Gateway Out9/1
  Delay80/1 -> Gateway Out8/1
  Gateway Out6/1 -> Scope1/1
  Gateway Out7/1 -> Scope1/2
  Gateway Out4/1 -> Scope1/3
  Gateway Out5/1 -> Scope1/4
  Slice1/1 -> Gateway Out5/1
  Delay81/1 -> Slice1/1
  Delay82/1 -> Gateway Out4/1
  Delay83/1 -> Gateway Out7/1
  Delay84/1 -> Gateway Out6/1
  [wr_en] -> [wr_en_0]
  [wr_en] -> [wr_en_1]
  [wr_addr] -> [wr_addr_1]
  [rd_en] -> [rd_en_1]
  [rd_addr] -> [rd_addr_0]
  [rd_tag] -> [rd_tag_1]
  Delay4/1 -> [hmc_d256_1]
  [hmc_d256_1_tmp] -> Delay4/1
  [hmc_tag_1_tmp] -> Delay17/1
  Delay17/1 -> [hmc_tag_1]
  [hmc_dv_1_tmp] -> Delay18/1
  Delay18/1 -> [hmc_dv_1]
  [hmc_d256_0] -> Delay9/1
  [hmc_dv_1] -> Delay11/1
  Delay11/1 -> obuf/5(dv1)
  [hmc_tag_1] -> Delay12/1
  Delay12/1 -> obuf/6(tag1)
  Delay13/1 -> obuf/7(din1)
  [hmc_d256_1] -> Delay13/1
  [ct_tvg_en] -> Subsystem1/3(tvg_sel)
  Delay25/1 -> Delay63/1
  Delay26/1 -> Delay48/1, Delay21/2, Delay22/2, Delay66/1
  Delay27/1 -> Delay22/1, Relational1/2, Delay72/1
  Delay28/1 -> Delay73/1
  Delay29/1 -> Delay85/1
  Delay40/1 -> Delay86/1
  Delay61/1 -> Delay94/1
  Delay62/1 -> Delay95/1
  Subsystem1/1(dout) -> Relational1/1, Delay21/1
  Delay72/1 -> bus_expand12/1(bus_in), bus_expand3/1(bus_in), Slice34/1, out_d256/1
  Delay73/1 -> Reinterpret1/1, pipeline64/1(d), pipeline17/1(d), pipeline43/1(d), pkt_start/1, Gateway Out22/1, Gateway Out14/1
  Delay85/1 -> [raw_freq_ctr_g]
  Delay86/1 -> pipeline65/1(d), pipeline61/1(d), Relational19/1, pipeline46/1(d), Gateway Out15/1, freq_id/1
  Delay94/1 -> x_index/1, Relational20/1, pipeline45/1(d), pipeline59/1(d), pipeline67/1(d), pipeline62/1(d), Gateway Out23/1, Gateway Out89/1
  Delay95/1 -> pipeline44/1(d), pipeline63/1(d), x_pkt_index/1, Gateway Out90/1
  Relational1/1 -> Gateway Out88/1, tvg_error/1
  Delay/1 -> Subsystem1/1(rst), Delay25/1
  Gateway Out12/1 -> Scope3/1
  Gateway Out13/1 -> Scope3/2
  Gateway Out14/1 -> Scope3/3
  Gateway Out15/1 -> Scope3/4
  Gateway Out20/1 -> Scope5/1
  Gateway Out21/1 -> Scope5/2
  Gateway Out22/1 -> Scope5/3
  Gateway Out23/1 -> Scope5/4
  Gateway Out33/1 -> Scope9/1
  Gateway Out34/1 -> Scope9/2
  Gateway Out35/1 -> Scope9/3
  Gateway Out36/1 -> Scope9/4
  Gateway Out41/1 -> Scope11/1
  Gateway Out42/1 -> Scope11/2
  Gateway Out43/1 -> Scope11/3
  Gateway Out44/1 -> Scope11/4
  Gateway Out45/1 -> Scope13/1
  Gateway Out46/1 -> Scope13/2
  Gateway Out47/1 -> Scope13/3
  Gateway Out48/1 -> Scope13/4
  Gateway Out49/1 -> Scope12/1
  Gateway Out50/1 -> Scope12/2
  Gateway Out51/1 -> Scope12/3
  Gateway Out52/1 -> Scope12/4
  Gateway Out37/1 -> Scope16/1
  Gateway Out38/1 -> Scope16/2
  Gateway Out39/1 -> Scope16/3
  Gateway Out40/1 -> Scope16/4
  Gateway Out53/1 -> Scope10/1
  Gateway Out54/1 -> Scope10/2
  Gateway Out55/1 -> Scope10/3
  Gateway Out56/1 -> Scope10/4
  Gateway Out57/1 -> Scope15/1
  Gateway Out58/1 -> Scope15/2
  Gateway Out59/1 -> Scope15/3
  Gateway Out60/1 -> Scope15/4
  Gateway Out61/1 -> Scope14/1
  Gateway Out62/1 -> Scope14/2
  Gateway Out63/1 -> Scope14/3
  Gateway Out64/1 -> Scope14/4
  bus_expand/1(msb_out16) -> Gateway Out35/1, Relational6/1
  bus_expand1/1(msb_out16) -> Gateway Out91/1, Gateway Out36/1, Relational6/2
  Relational6/1 -> Gateway Out34/1
  Relational7/1 -> Gateway Out42/1
  bus_expand/2(out15) -> Gateway Out43/1, Relational7/1
  bus_expand1/2(out15) -> Gateway Out44/1, Relational7/2
  bus_expand1/3(out14) -> Relational8/2, Gateway Out48/1
  bus_expand/3(out14) -> Gateway Out47/1, Relational8/1
  Relational8/1 -> Gateway Out46/1
  Relational9/1 -> Gateway Out50/1
  bus_expand/4(out13) -> Gateway Out51/1, Relational9/1
  bus_expand1/4(out13) -> Gateway Out52/1, Relational9/2
  Relational10/1 -> Gateway Out38/1
  bus_expand/5(out12) -> Gateway Out39/1, Relational10/1
  bus_expand1/5(out12) -> Relational10/2, Gateway Out40/1
  Relational11/1 -> Gateway Out54/1
  bus_expand/6(out11) -> Gateway Out55/1, Relational11/1
  bus_expand1/6(out11) -> Relational11/2, Gateway Out56/1
  Relational12/1 -> Gateway Out58/1
  bus_expand/7(out10) -> Gateway Out59/1, Relational12/1
  bus_expand1/7(out10) -> Gateway Out60/1, Relational12/2
  Relational13/1 -> Gateway Out62/1
  bus_expand/8(out9) -> Gateway Out63/1, Relational13/1
  Gateway Out73/1 -> Scope20/1
  Gateway Out74/1 -> Scope20/2
  Gateway Out75/1 -> Scope20/3
  Gateway Out76/1 -> Scope20/4
  Relational14/1 -> Gateway Out74/1, Gateway Out16/1
  bus_expand1/16(lsb_out1) -> Gateway Out19/1, Relational18/1, Gateway Out76/1, Relational14/2
  bus_expand/16(lsb_out1) -> Delay23/1, Gateway Out75/1, Relational14/1
  Delay21/1 -> bus_expand/1(bus_in)
  Delay22/1 -> bus_expand1/1(bus_in)
  Gateway Out24/1 -> Scope6/1
  Gateway Out25/1 -> Scope6/2
  Gateway Out26/1 -> Scope6/3
  Gateway Out27/1 -> Scope6/4
  Relational2/1 -> Gateway Out25/1
  Delay48/1 -> Gateway Out28/1, Gateway Out32/1, Gateway Out68/1, Gateway Out72/1, Gateway Out80/1, Gateway Out84/1, Delay23/2, Gateway Out17/1, Counter1/2, Gateway Out73/1, Gateway Out24/1, Gateway Out61/1, Gateway Out57/1, Gateway Out53/1, Gateway Out37/1, Gateway Out49/1, Gateway Out45/1, Gateway Out41/1, Gateway Out33/1
  bus_expand/9(out8) -> Gateway Out26/1, Relational2/1
  bus_expand1/9(out8) -> Gateway Out27/1, Relational2/2
  Gateway Out28/1 -> Scope7/1
  Gateway Out29/1 -> Scope7/2
  Gateway Out30/1 -> Scope7/3
  Gateway Out31/1 -> Scope7/4
  Relational3/1 -> Gateway Out29/1
  bus_expand/10(out7) -> Gateway Out30/1, Relational3/1
  bus_expand1/10(out7) -> Gateway Out31/1, Relational3/2
  Gateway Out32/1 -> Scope8/1
  Gateway Out65/1 -> Scope8/2
  Gateway Out66/1 -> Scope8/3
  Gateway Out67/1 -> Scope8/4
  Relational4/1 -> Gateway Out65/1
  bus_expand1/8(out9) -> Gateway Out64/1, Relational13/2
  bus_expand1/11(out6) -> Gateway Out67/1, Relational4/2
  bus_expand/11(out6) -> Gateway Out66/1, Relational4/1
  Gateway Out68/1 -> Scope17/1
  Gateway Out69/1 -> Scope17/2
  Gateway Out70/1 -> Scope17/3
  Gateway Out71/1 -> Scope17/4
  Gateway Out72/1 -> Scope4/1
  Gateway Out77/1 -> Scope4/2
  Gateway Out78/1 -> Scope4/3
  Gateway Out79/1 -> Scope4/4
  Relational5/1 -> Gateway Out69/1
  bus_expand/12(out5) -> Gateway Out70/1, Relational5/1
  bus_expand1/12(out5) -> Gateway Out71/1, Relational5/2
  Relational15/1 -> Gateway Out77/1
  bus_expand/13(out4) -> Gateway Out78/1, Relational15/1
  bus_expand1/13(out4) -> Gateway Out79/1, Relational15/2
  Gateway Out80/1 -> Scope18/1
  Gateway Out81/1 -> Scope18/2
  Gateway Out82/1 -> Scope18/3
  Gateway Out83/1 -> Scope18/4
  Relational16/1 -> Gateway Out81/1
  bus_expand/14(out3) -> Gateway Out82/1, Relational16/1
  bus_expand1/14(out3) -> Gateway Out83/1, Relational16/2
  Gateway Out84/1 -> Scope19/1
  Gateway Out85/1 -> Scope19/2
  Gateway Out86/1 -> Scope19/3
  Gateway Out87/1 -> Scope19/4
  Relational17/1 -> Gateway Out85/1
  bus_expand/15(out2) -> Gateway Out86/1, Relational17/1
  bus_expand1/15(out2) -> Gateway Out87/1, Relational17/2
  Gateway Out16/1 -> Scope21/1
  Gateway Out17/1 -> Scope21/2
  Gateway Out18/1 -> Scope21/3
  Gateway Out19/1 -> Scope21/4
  Relational18/1 -> Counter1/1
  Delay23/1 -> Relational18/2
  Counter1/1 -> Gateway Out18/1
  [wr_addr_0] -> pipeline/1(d)  "WR_addr"
  [wr_d256_0] -> pipeline1/1(d)
  [rd_addr_0] -> pipeline2/1(d)  "RD_rdaddr"
  [rd_tag_0] -> pipeline3/1(d)  "RD_tag"
  hmc1/11 -> [hmc_ok1]
  hmc/11 -> [hmc_ok0]
  Gateway Out88/1 -> Scope3/5
  Gateway Out89/1 -> Scope3/6
  Gateway Out90/1 -> Scope3/7
  Gateway Out91/1 -> Scope3/8
  [hmc_rd_rdy_0] -> Subsystem2/2(In2)
  Subsystem4/2(out1) -> status2/2(out_fifo_full_err_cnt)
  [obuf_proc_err_miss_0_g] -> Subsystem4/4(in2)
  Constant13/1 -> Subsystem4/3(in1)
  [rd_go_err_g] -> Subsystem5/5(in3)
  [ct_bank_error_g0] -> Subsystem5/2(in0)
  [ct_bank_error_g1] -> Subsystem5/3(in1)
  Subsystem5/3(out2) -> status1/3(out_obuff_bank_err_cnt)
  Subsystem5/2(out1) -> status1/2(out_bank_err_cnt_pol1)
  [hmc_ok0] -> Inverter3/1
  Subsystem5/4(out3) -> status1/4(out_rd_go_err_cnt)
  Inverter3/1 -> Subsystem3/2(in0)
  [cthmc_sync_err_g0] -> Subsystem4/2(in0)
  [hmc_ok1] -> Inverter4/1
  [cnt_rst] -> Subsystem2/1(In1)
  Subsystem2/2(Out2) -> status0/2(out_hmc_overflow_err_cnt_pol1)
  Subsystem2/1(Out1) -> status0/1(out_hmc_overflow_err_cnt_pol0)
  [cnt_rst] -> Subsystem3/1(rst)
  Inverter4/1 -> Subsystem3/3(in1)
  Subsystem4/4(out3) -> status2/4(out_reorder_missing_err_cnt1)
  Subsystem4/1(out0) -> status2/1(out_sync_in_err_cnt)
  Subsystem4/3(out2) -> status2/3(out_reorder_missing_err_cnt)
  [hmc_wr_rdy_1] -> Subsystem2/5(In5)
  Subsystem3/2(out1) -> status0/4(out_hmc_err_cnt1)
  Subsystem3/1(out0) -> status0/3(out_hmc_err_cnt0)
  [cnt_rst] -> Subsystem4/1(rst)
  Subsystem5/1(out0) -> status1/1(out_bank_err_cnt_pol0)
  [cnt_rst] -> Subsystem5/1(rst)
  [hmc_wr_rdy_0] -> Subsystem2/3(In3)
  [hmc_rd_rdy_1] -> Subsystem2/4(In4)
  [obuf_ct_addr_err_g] -> Subsystem5/4(in2)
  [obuf_proc_err_miss_1_g] -> Subsystem4/5(in3)
  [hmc_ok0] -> Inverter5/1
  [hmc_ok1] -> Inverter7/1
  Inverter5/1 -> Logical4/1
  Inverter7/1 -> Logical4/2
  Inverter22/1 -> Logical4/3
  Inverter23/1 -> Logical4/4
  Inverter1/1 -> Logical4/5
  Inverter2/1 -> Logical4/6
  we_delay6/1(q) -> snap_tag/1(in_sync)
  From8/1 -> time_gen_1/5(rd_en)
  we_delay4/1(q) -> snap_tag/3(in_time)
  time_gen_1/2(rd_dvalid) -> Logical3/1, we_delay5/1(d)
  Concat1/1 -> time_gen_1/6(rd_misc_in)
  From289/1 -> snap_tag/9(arm)
  From12/1 -> Delay20/1
  From255/1 -> time_gen_1/1(wr_sync_in)
  From274/1 -> time_gen_1/2(wr_en)
  we_delay2/1(q) -> snap_tag/5(in_data)
  we_delay7/1(q) -> snap_tag/7(we)
  we_delay5/1(q) -> snap_tag/2(in_dv)
  From_pfb_d3/1 -> time_gen_1/3(wr_val_in)
  From10/1 -> spectrum_ctr1/1
  From9/1 -> Concat1/1
  spectrum_ctr1/1 -> Concat1/2
  time_gen_1/4(rd_misc_out) -> bus_expand9/1(bus_in)
  we_delay3/1(q) -> snap_tag/4(in_tag)
  From/1 -> Delay19/1
  Delay19/1 -> Reinterpret/1
  bus_expand9/1(msb_out3) -> we_delay3/1(d)
  bus_expand9/2(out2) -> we_delay2/1(d)
  Reinterpret/1 -> Concat1/3
  we_delay1/1(q) -> snap_tag/6(in_rd_rdy)
  bus_expand9/3(lsb_out1) -> we_delay1/1(d)
  Delay20/1 -> time_gen_1/4(rd_sync_in)
  Logical3/1 -> we_delay7/1(d)
  Logical6/1 -> we_delay14/1(d)
  From_rd_en_2/1 -> Logical6/1, we_delay21/1(d)
  we_delay14/1(q) -> snap_hmc/15(we)
  From40/1 -> snap_hmc/17(arm)
  From60/1 -> we_delay22/1(d)
  From_rd_addr_2/1 -> we_delay20/1(d)
  From_rd_tag0_2/1 -> we_delay19/1(d)
  From_wr_addr_2/1 -> we_delay18/1(d)
  From_wr_en_2/1 -> we_delay17/1(d)
  From_wr_d256_2/1 -> spectrum_ctr5/1
  spectrum_ctr5/1 -> we_delay16/1(d)
  From42/1 -> we_delay13/1(d)
  From56/1 -> we_delay12/1(d)
  From7/1 -> spectrum_ctr6/1
  From43/1 -> we_delay10/1(d)
  From44/1 -> we_delay9/1(d)
  From61/1 -> we_delay8/1(d)
  spectrum_ctr6/1 -> we_delay11/1(d)
  we_delay8/1(q) -> snap_hmc/14(in_hmc_ok)
  we_delay9/1(q) -> snap_hmc/13(in_hmc_rd_rdy)
  we_delay10/1(q) -> snap_hmc/12(in_hmc_wr_rdy)
  we_delay11/1(q) -> snap_hmc/11(in_hmc_data)
  we_delay12/1(q) -> snap_hmc/10(in_hmc_tag)
  we_delay13/1(q) -> snap_hmc/9(in_hmc_dv)
  we_delay16/1(q) -> snap_hmc/7(in_wr_data)
  we_delay17/1(q) -> snap_hmc/6(in_wr_en)
  we_delay18/1(q) -> snap_hmc/5(in_wr_addr)
  we_delay19/1(q) -> snap_hmc/4(in_rd_tag)
  we_delay20/1(q) -> snap_hmc/3(in_rd_addr)
  we_delay21/1(q) -> snap_hmc/2(in_dv)
  we_delay22/1(q) -> snap_hmc/1(in_sync)
  edge_detect3/1(out) -> snap_hmc/16(trig)
  edge_detect2/1(out) -> snap_tag/8(trig)
  we_delay24/1(q) -> sync_time_hmc_out_lsw/1(out_lsw)
  time_gen_1/3(rd_val_out) -> spectrum_ctr7/1, spectrum_ctr8/1, we_delay4/1(d)
  time_gen_1/1(rd_sync_out) -> edge_detect6/1(in), we_delay6/1(d), Logical3/2, edge_detect2/1(in)
  spectrum_ctr8/1 -> Register5/1
  Register5/1 -> we_delay24/1(d)
  From169/1 -> Register5/2, Register6/2
  edge_detect6/1(out) -> Register5/3, Register6/3
  Register6/1 -> we_delay23/1(d)
  we_delay23/1(q) -> sync_time_hmc_out_msw/1(out_msw)
  spectrum_ctr7/1 -> Register6/1
  spectrum_ctr10/1 -> Register2/1
  we_delay27/1(q) -> sync_time_hmc_in_msw/1(out_msw)
  Register2/1 -> we_delay27/1(d)
  edge_detect5/1(out) -> Register2/3, Register1/3
  From28/1 -> Register2/2, Register1/2
  Register1/1 -> we_delay28/1(d)
  spectrum_ctr11/1 -> Register1/1
  time_gen_3/1(rd_sync_out) -> edge_detect5/1(in)
  time_gen_3/3(rd_val_out) -> spectrum_ctr11/1, spectrum_ctr10/1
  we_delay28/1(q) -> sync_time_hmc_in_lsw/1(out_lsw)
  From72/1 -> time_gen_3/4(rd_sync_in)
  From_pfb_d1/1 -> time_gen_3/3(wr_val_in)
  From71/1 -> time_gen_3/2(wr_en)
  From66/1 -> time_gen_3/1(wr_sync_in)
  From23/1 -> time_gen_3/5(rd_en)
  Constant14/1 -> time_gen_3/6(rd_misc_in)
  we_delay53/1(q) -> sync_lat_ct_in_free/1(out_count)
  Register36/1 -> we_delay53/1(d)
  edge_detect28/1(out) -> Register36/3
  From76/1 -> edge_detect28/1(in)
  Counter45/1 -> Register36/1
  we_delay25/1(q) -> sync_lat_hmc_addgen/1(out_count)
  From78/1 -> Counter3/1, Register4/2
  we_delay26/1(q) -> sync_lat_hmc_addgen_free/1(out_count)
  Register4/1 -> we_delay26/1(d)
  edge_detect4/1(out) -> Register4/3
  From84/1 -> edge_detect4/1(in)
  Counter3/1 -> Register4/1
  Counter5/1 -> Register8/1
  edge_detect7/1(out) -> Register8/3
  Register8/1 -> we_delay30/1(d)
  we_delay30/1(q) -> sync_lat_hmc_free/1(out_count)
  From88/1 -> Register8/2, Counter5/1
  we_delay29/1(q) -> sync_lat_hmc/1(out_count)
  edge_detect40/1(out) -> Register49/3
  Slice34/1 -> Register49/1
  we_delay66/1(q) -> sync_latch_hmc/1(out_count)
  Register49/1 -> we_delay66/1(d)
  edge_detect8/1(out) -> Register9/3
  Slice2/1 -> Register9/1
  we_delay31/1(q) -> sync_latch_ct_in/1(out_count)
  Register9/1 -> we_delay31/1(d)
  From89/1 -> edge_detect8/1(in)
  From90/1 -> Slice2/1
  edge_detect9/1(out) -> Register10/3
  Slice3/1 -> Register10/1
  we_delay32/1(q) -> sync_latch_hmc_addgen/1(out_count)
  Register10/1 -> we_delay32/1(d)
  From91/1 -> Register10/2
  From92/1 -> edge_detect9/1(in)
  From97/1 -> Slice3/1
  From99/1 -> edge_detect10/1(in)
  From98/1 -> Register11/2
  Register11/1 -> we_delay33/1(d)
  we_delay33/1(q) -> sync_latch_hmc_rdadd/1(out_count)
  From100/1 -> Register11/1
  edge_detect10/1(out) -> Register11/3
  edge_detect11/1(out) -> Register12/3
  From102/1 -> Register12/1
  we_delay35/1(q) -> sync_latch_hmc_wradd/1(out_count)
  Register12/1 -> we_delay35/1(d)
  From104/1 -> Register12/2
  From105/1 -> edge_detect11/1(in)
  From107/1 -> edge_detect12/1(in)
  From106/1 -> Register13/2
  Register13/1 -> we_delay36/1(d)
  we_delay36/1(q) -> sync_latch_hmc_tag/1(out_count)
  From101/1 -> Register13/1
  edge_detect12/1(out) -> Register13/3
  obuf/1(out_sync) -> gen_freq_calc/1(sync), edge_detect14/1(in), Register15/2, edge_detect13/1(in), Delay/1
  From108/1 -> Register14/2
  Register14/1 -> we_delay39/1(d)
  we_delay39/1(q) -> sync_latch_hmc_reord/1(out_count)
  Slice7/1 -> Register14/1
  edge_detect14/1(out) -> Register14/3
  Counter7/1 -> Register16/1
  edge_detect13/1(out) -> Register16/3
  Register16/1 -> we_delay38/1(d)
  we_delay38/1(q) -> sync_lat_hmc_reord_free/1(out_count)
  From118/1 -> Register16/2, Counter7/1
  edge_detect51/1(out) -> Register62/3
  Register24/1 -> edge_detect51/1(in), Logical29/1
  Counter33/1 -> Register62/1
  Logical29/1 -> Counter33/2
  Register62/1 -> we_delay25/1(d)
  From85/1 -> Logical29/2
  From77/1 -> Register62/2, Counter33/1, Register24/1, Register24/3
  From83/1 -> Register24/2
  edge_detect15/1(out) -> Register17/3
  Register3/1 -> edge_detect15/1(in), Logical7/1
  Counter2/1 -> Register17/1
  Logical7/1 -> Counter2/2
  Register17/1 -> we_delay34/1(d)
  From75/1 -> Register3/2
  we_delay34/1(q) -> sync_lat_ct_in/1(out_count)
  edge_detect16/1(out) -> Register18/3
  Register15/1 -> edge_detect16/1(in), Logical12/1
  Counter6/1 -> Register18/1
  Logical12/1 -> Counter6/2
  Register18/1 -> we_delay37/1(d)
  From115/1 -> Logical12/2
  From103/1 -> Register18/2, Counter6/1, Register15/1, Register15/3
  obuf/3(out_d) -> Slice7/1, Delay10/1
  we_delay37/1(q) -> sync_lat_hmc_reord/1(out_count)
  edge_detect17/1(out) -> Register19/3
  Register7/1 -> edge_detect17/1(in), Logical9/1
  Counter4/1 -> Register19/1
  Logical9/1 -> Counter4/2
  Register19/1 -> we_delay29/1(d)
  From_rd_en_3/1 -> Logical9/2
  From86/1 -> Register19/2, Counter4/1, Register7/1, Register7/3, Register49/2
  From112/1 -> edge_detect3/1(in), Logical6/2, we_delay15/1(d)
  we_delay15/1(q) -> snap_hmc/8(in_rd_arm)
  bus_expand3/1(msb_out16) -> bus_expand2/1(bus_in)
  bus_expand2/1(msb_out2) -> pipeline54/1(d)
  bus_expand4/1(msb_out2) -> pipeline53/1(d)
  bus_expand5/1(msb_out2) -> pipeline52/1(d)
  bus_expand6/1(msb_out2) -> pipeline51/1(d)
  bus_expand7/1(msb_out2) -> pipeline50/1(d)
  bus_expand8/1(msb_out2) -> pipeline49/1(d)
  bus_expand10/1(msb_out2) -> pipeline48/1(d)
  bus_expand11/1(msb_out2) -> pipeline47/1(d)
  bus_expand3/3(out14) -> bus_expand4/1(bus_in)
  bus_expand3/5(out12) -> bus_expand5/1(bus_in)
  bus_expand3/7(out10) -> bus_expand6/1(bus_in)
  bus_expand3/9(out8) -> bus_expand7/1(bus_in)
  bus_expand3/11(out6) -> bus_expand8/1(bus_in)
  bus_expand3/13(out4) -> bus_expand10/1(bus_in)
  bus_expand3/15(out2) -> bus_expand11/1(bus_in)
  pipeline21/1(q) -> ss_ct2/5(in_pkt_start)
  pipeline22/1(q) -> ss_ct2/4(in_x_pkt)
  pipeline23/1(q) -> ss_ct2/3(in_x_idx)
  pipeline24/1(q) -> ss_ct2/2(in_freq_id)
  pipeline26/1(q) -> ss_ct1/16(trig)
  pipeline27/1(q) -> ss_ct1/15(we)
  pipeline28/1(q) -> ss_ct1/14(in_sync)
  pipeline29/1(q) -> ss_ct1/13(in_dv)
  pipeline30/1(q) -> ss_ct1/12(in_pkt_start)
  pipeline31/1(q) -> ss_ct1/11(in_x_pkt)
  pipeline32/1(q) -> ss_ct1/10(in_x_idx)
  pipeline33/1(q) -> ss_ct1/9(in_freq_id)
  pipeline34/1(q) -> ss_ct1/8(in_f7_re)
  pipeline35/1(q) -> ss_ct1/7(in_f6_re)
  pipeline36/1(q) -> ss_ct1/6(in_f5_re)
  pipeline37/1(q) -> ss_ct1/5(in_f4_re)
  pipeline38/1(q) -> ss_ct1/4(in_f3_re)
  pipeline39/1(q) -> ss_ct1/3(in_f2_re)
  pipeline40/1(q) -> ss_ct1/2(in_f1_re)
  pipeline41/1(q) -> ss_ct1/1(in_f0_re)
  Constant15/1 -> freq_trig_thresh/1(sim_1)
  xidx_trig_thresh/1(in_threshold) -> pipeline15/1(d)
  freq_trig_thresh/1(in_threshold) -> pipeline14/1(d)
  Constant67/1 -> xidx_trig_thresh/1(sim_1)
  pipeline14/1(q) -> Relational19/2
  Mux1/1 -> Delay74/1, pipeline26/1(d), pipeline28/1(d)
  Constant16/1 -> ct_trig_sel/1(sim_1)
  Delay66/1 -> out_dv/1, Gateway Out21/1, Gateway Out13/1, pipeline42/1(d), pipeline19/1(d), pipeline55/1(d), pipeline72/1(d), pipeline70/1(d), pipeline68/1(d), pipeline66/1(d)
  pipeline15/1(q) -> Relational20/2
  pipeline16/1(q) -> Mux1/1
  Delay63/1 -> pipeline18/1(d), edge_detect7/1(in), Register7/2, edge_detect40/1(in), out_sync/1, Gateway Out12/1, Gateway Out20/1
  Relational20/1 -> Mux1/3
  ct_trig_sel/1(in_sel) -> pipeline16/1(d)
  pipeline17/1(q) -> Mux1/4
  Relational19/1 -> Mux1/5
  pipeline18/1(q) -> Mux1/2
  pipeline19/1(q) -> Delay58/1
  pipeline42/1(q) -> Delay24/1
  pipeline43/1(q) -> Delay30/1
  pipeline44/1(q) -> Delay31/1
  pipeline45/1(q) -> Delay32/1
  pipeline46/1(q) -> Delay37/1
  pipeline47/1(q) -> Delay38/1
  pipeline49/1(q) -> Delay50/1
  pipeline48/1(q) -> Delay49/1
  pipeline52/1(q) -> Delay55/1
  pipeline50/1(q) -> Delay52/1
  pipeline53/1(q) -> Delay56/1
  pipeline51/1(q) -> Delay53/1
  pipeline54/1(q) -> Delay57/1
  Delay24/1 -> pipeline29/1(d)
  Delay30/1 -> pipeline30/1(d)
  Delay31/1 -> pipeline31/1(d)
  Delay32/1 -> pipeline32/1(d)
  Delay37/1 -> pipeline33/1(d)
  Delay38/1 -> pipeline34/1(d)
  Delay49/1 -> pipeline35/1(d)
  Delay50/1 -> pipeline36/1(d)
  Delay52/1 -> pipeline37/1(d)
  Delay53/1 -> pipeline38/1(d)
  Delay55/1 -> pipeline39/1(d)
  Delay56/1 -> pipeline40/1(d)
  Delay57/1 -> pipeline41/1(d)
  Delay58/1 -> pipeline27/1(d)
  Delay69/1 -> Delay92/1
  Delay68/1 -> Delay91/1
  Delay67/1 -> Delay88/1
  Delay59/1 -> Delay87/1
  Delay71/1 -> Delay76/1
  pipeline20/1(q) -> ss_ct2/7(in_trig)
  pipeline56/1(q) -> ss_ct2/9(trig)
  pipeline57/1(q) -> ss_ct2/8(we)
  pipeline58/1(q) -> ss_ct2/6(in_dv)
  pipeline60/1(q) -> Delay69/1
  pipeline61/1(q) -> Delay68/1
  pipeline62/1(q) -> Delay67/1
  pipeline63/1(q) -> Delay59/1
  pipeline64/1(q) -> Delay71/1
  pipeline65/1(q) -> data_change/1(data)
  pipeline66/1(q) -> data_change/2(dv)
  pipeline68/1(q) -> data_change1/2(dv)
  pipeline67/1(q) -> data_change1/1(data)
  Mux2/1 -> pipeline58/1(d), pipeline57/1(d), pipeline74/1(d)
  ct2_dv_sel/1(in_sel) -> pipeline69/1(d)
  Constant17/1 -> ct2_dv_sel/1(sim_1)
  pipeline69/1(q) -> Mux2/1
  Delay76/1 -> pipeline21/1(d)
  Delay87/1 -> pipeline22/1(d)
  Delay88/1 -> pipeline23/1(d)
  Delay91/1 -> pipeline24/1(d)
  Delay92/1 -> pipeline25/1(d)
  pipeline70/1(q) -> Delay97/1
  Delay97/1 -> Mux2/4
  pipeline71/1(q) -> data_change2/1(data)
  pipeline72/1(q) -> data_change2/2(dv)
  Reinterpret1/1 -> pipeline71/1(d)
  Counter8/1 -> pipeline73/1(d)
  pipeline73/1(q) -> ct2_dv_cnt/1(out_cnt)
  pipeline74/1(q) -> Counter8/2
  Logical17/1 -> Counter8/1
  [cnt_rst] -> Logical17/1
  Delay74/1 -> pipeline20/1(d), pipeline56/1(d), Logical17/2
  data_change/1(trig) -> Logical13/2, Mux2/2
  data_change1/1(trig) -> Mux2/3
  data_change2/1(trig) -> Mux2/5
  pipeline25/1(q) -> ss_ct2/1(in_data0)
  bus_expand12/1(msb_out8) -> Convert/1
  Constant18/1 -> xeng_match/1(sim_1)
  match/1(Out1) -> Logical13/1, Mux2/6
  pipeline55/1(q) -> match/1(dv)
  pipeline59/1(q) -> match/2(data)
  xeng_match/1(in_val) -> pipeline75/1(d)
  pipeline75/1(q) -> match/3(match_value)
  Logical13/1 -> Mux2/7
  Convert/1 -> pipeline60/1(d)
